simulink model "PV_WIND_BESS_ISLAND_R1"  (R2023b)
settings: Solver=ode14x  StartTime=0.0  StopTime=3.2  FixedStep=25e-6  MaxStep=1e-5  RelTol=1e-3
InitFcn:
  | setup_v2_paths;init_grid_supported_integration;run(which('init_bess_vsm_r10.m'));
undefined symbols (not defined in the file): Base, Control, Converter, DiscIntNeverNeededParam, Drive, Filter, G, PMSG, V2, Wind
libraries: nesl_utility x51, ee_lib x44, fl_lib x25, simulink x6
(part 4 of 4)

== system PV_WIND_BESS_ISLAND_R1/PV Resource/04 Local GFL Control/03 Vdc and Q to current reference/DC Voltage PI ==
  error : Inport
  Integral Derivative : Sum
  Integrator : DiscreteIntegrator  SampleTime=100e-6  ICPrevOutput=DiscIntNeverNeededParam  ICPrevScaledInput=DiscIntNeverNeededParam
  Kaw : Gain  Gain=V2.PV.dynamic.dc_Kaw
  Ki : Gain  Gain=V2.PV.dynamic.dc_Ki_ApVs
  Kp : Gain  Gain=V2.PV.dynamic.dc_Kp_ApV
  Limit : Saturate  UpperLimit=V2.PV.control.Ilimit_peak_A  LowerLimit=-V2.PV.control.Ilimit_peak_A
  Tracking Error : Sum  Inputs=+-
  Unsaturated : Sum
  output : Outport
  wires:
  Tracking Error/1 -> Kaw/1
  Limit/1 -> Tracking Error/1, output/1
  Unsaturated/1 -> Tracking Error/2, Limit/1
  Kp/1 -> Unsaturated/1
  Integrator/1 -> Unsaturated/2
  Integral Derivative/1 -> Integrator/1
  Kaw/1 -> Integral Derivative/2
  Ki/1 -> Integral Derivative/1
  error/1 -> Ki/1, Kp/1

== system PV_WIND_BESS_ISLAND_R1/Wind Resource/02 PMSG dq Machine and Average MSC/01 Torque and Current References/Dispatch Torque Limit ==
  In1 : Inport
  In2 : Inport  Port=2
  Dispatch Inputs : Mux
  Dispatch Torque Cap : Fcn  Expr=0.5*(u(1)+u(2)/u(3)-abs(u(1)-u(2)/u(3)))*u(4)
  Speed Floor : Saturate  UpperLimit=inf  LowerLimit=PMSG.speed_floor_rad_s
  Out1 : Outport
  wires:
  Speed Floor/1 -> Dispatch Inputs/3
  In2/1 -> Dispatch Inputs/1
  Dispatch Inputs/1 -> Dispatch Torque Cap/1
  [WIND_R4__DISPATCH_W] -> Dispatch Inputs/2
  Dispatch Torque Cap/1 -> Out1/1
  In1/1 -> Speed Floor/1
  [WIND_R4__ENABLE] -> Dispatch Inputs/4

== system PV_WIND_BESS_ISLAND_R1/Wind Resource/03 DC Link and Two-Level GSC/Converter AC Measurement/Line Voltage Calculation ==
  Vabc : Inport
  Separate abc : Demux  Outputs=3
  Vab = Va - Vb : Sum  Inputs=+-
  Vab Vbc Vca : Mux  Inputs=3
  Vbc = Vb - Vc : Sum  Inputs=+-
  Vca = Vc - Va : Sum  Inputs=+-
  Vll : Outport
  wires:
  Vabc/1 -> Separate abc/1
  Separate abc/1 -> Vab = Va - Vb/1, Vca = Vc - Va/2
  Separate abc/2 -> Vab = Va - Vb/2, Vbc = Vb - Vc/1
  Separate abc/3 -> Vbc = Vb - Vc/2, Vca = Vc - Va/1
  Vab = Va - Vb/1 -> Vab Vbc Vca/1
  Vbc = Vb - Vc/1 -> Vab Vbc Vca/2
  Vca = Vc - Va/1 -> Vab Vbc Vca/3
  Vab Vbc Vca/1 -> Vll/1  "Vll_inv"

== system PV_WIND_BESS_ISLAND_R1/Wind Resource/04 GFL Control and SPWM/01 Measurements and dq/Current alpha beta to dq ==
  alpha beta : Inport
  theta : Inport  Port=2
  Separate alpha beta : Demux  Outputs=2
  alpha cos : Product
  alpha sin : Product
  beta cos : Product
  beta sin : Product
  cos theta : Trigonometry  Operator=cos
  d = alpha cos + beta sin : Sum
  dq vector : Mux  Inputs=2
  q = -alpha sin + beta cos : Sum  Inputs=-+
  sin theta : Trigonometry
  dq : Outport
  wires:
  alpha beta/1 -> Separate alpha beta/1
  theta/1 -> cos theta/1, sin theta/1
  Separate alpha beta/1 -> alpha cos/1, alpha sin/1
  cos theta/1 -> alpha cos/2, beta cos/2
  Separate alpha beta/2 -> beta sin/1, beta cos/1
  sin theta/1 -> beta sin/2, alpha sin/2
  alpha cos/1 -> d = alpha cos + beta sin/1
  beta sin/1 -> d = alpha cos + beta sin/2
  alpha sin/1 -> q = -alpha sin + beta cos/1
  beta cos/1 -> q = -alpha sin + beta cos/2
  d = alpha cos + beta sin/1 -> dq vector/1
  q = -alpha sin + beta cos/1 -> dq vector/2
  dq vector/1 -> dq/1

== system PV_WIND_BESS_ISLAND_R1/Wind Resource/04 GFL Control and SPWM/01 Measurements and dq/Voltage alpha beta to dq ==
  alpha beta : Inport
  theta : Inport  Port=2
  Separate alpha beta : Demux  Outputs=2
  alpha cos : Product
  alpha sin : Product
  beta cos : Product
  beta sin : Product
  cos theta : Trigonometry  Operator=cos
  d = alpha cos + beta sin : Sum
  dq vector : Mux  Inputs=2
  q = -alpha sin + beta cos : Sum  Inputs=-+
  sin theta : Trigonometry
  dq : Outport
  wires:
  alpha beta/1 -> Separate alpha beta/1
  theta/1 -> cos theta/1, sin theta/1
  Separate alpha beta/1 -> alpha cos/1, alpha sin/1
  cos theta/1 -> alpha cos/2, beta cos/2
  Separate alpha beta/2 -> beta sin/1, beta cos/1
  sin theta/1 -> beta sin/2, alpha sin/2
  alpha cos/1 -> d = alpha cos + beta sin/1
  beta sin/1 -> d = alpha cos + beta sin/2
  alpha sin/1 -> q = -alpha sin + beta cos/1
  beta cos/1 -> q = -alpha sin + beta cos/2
  d = alpha cos + beta sin/1 -> dq vector/1
  q = -alpha sin + beta cos/1 -> dq vector/2
  dq vector/1 -> dq/1

== system PV_WIND_BESS_ISLAND_R1/Wind Resource/04 GFL Control and SPWM/02 Synchronization SRF-PLL/PCC Voltage Prefilter ==
  abc raw : Inport
  Filtered abc : Mux  Inputs=3
  Phase A LPF : TransferFcn  Numerator=[2*pi*Control.PLL.VoltagePrefilterHz]  Denominator=[1 2*pi*Control.PLL.VoltagePrefilterHz]
  Phase B LPF : TransferFcn  Numerator=[2*pi*Control.PLL.VoltagePrefilterHz]  Denominator=[1 2*pi*Control.PLL.VoltagePrefilterHz]
  Phase C LPF : TransferFcn  Numerator=[2*pi*Control.PLL.VoltagePrefilterHz]  Denominator=[1 2*pi*Control.PLL.VoltagePrefilterHz]
  Separate abc : Demux  Outputs=3
  abc filtered : Outport
  wires:
  Separate abc/1 -> Phase A LPF/1
  Phase A LPF/1 -> Filtered abc/1
  Separate abc/2 -> Phase B LPF/1
  Phase B LPF/1 -> Filtered abc/2
  Separate abc/3 -> Phase C LPF/1
  Phase C LPF/1 -> Filtered abc/3
  abc raw/1 -> Separate abc/1
  Filtered abc/1 -> abc filtered/1

== system PV_WIND_BESS_ISLAND_R1/Wind Resource/04 GFL Control and SPWM/02 Synchronization SRF-PLL/Park Voltage ==
  alpha beta : Inport
  theta : Inport  Port=2
  Separate alpha beta : Demux  Outputs=2
  alpha cos : Product
  alpha sin : Product
  beta cos : Product
  beta sin : Product
  cos theta : Trigonometry  Operator=cos
  d = alpha cos + beta sin : Sum
  dq vector : Mux  Inputs=2
  q = -alpha sin + beta cos : Sum  Inputs=-+
  sin theta : Trigonometry
  dq : Outport
  wires:
  alpha beta/1 -> Separate alpha beta/1
  theta/1 -> cos theta/1, sin theta/1
  Separate alpha beta/1 -> alpha cos/1, alpha sin/1
  cos theta/1 -> alpha cos/2, beta cos/2
  Separate alpha beta/2 -> beta sin/1, beta cos/1
  sin theta/1 -> beta sin/2, alpha sin/2
  alpha cos/1 -> d = alpha cos + beta sin/1
  beta sin/1 -> d = alpha cos + beta sin/2
  alpha sin/1 -> q = -alpha sin + beta cos/1
  beta cos/1 -> q = -alpha sin + beta cos/2
  d = alpha cos + beta sin/1 -> dq vector/1
  q = -alpha sin + beta cos/1 -> dq vector/2
  dq vector/1 -> dq/1

== system PV_WIND_BESS_ISLAND_R1/Wind Resource/04 GFL Control and SPWM/03 DC Voltage and Current Reference/Park Voltage ==
  alpha beta : Inport
  theta : Inport  Port=2
  Separate alpha beta : Demux  Outputs=2
  alpha cos : Product
  alpha sin : Product
  beta cos : Product
  beta sin : Product
  cos theta : Trigonometry  Operator=cos
  d : Sum
  dq vector : Mux  Inputs=2
  q : Sum  Inputs=-+
  sin theta : Trigonometry
  dq : Outport
  wires:
  alpha beta/1 -> Separate alpha beta/1
  theta/1 -> cos theta/1, sin theta/1
  Separate alpha beta/1 -> alpha cos/1, alpha sin/1
  cos theta/1 -> alpha cos/2, beta cos/2
  Separate alpha beta/2 -> beta sin/1, beta cos/1
  sin theta/1 -> beta sin/2, alpha sin/2
  alpha cos/1 -> d/1
  beta sin/1 -> d/2
  alpha sin/1 -> q/1
  beta cos/1 -> q/2
  d/1 -> dq vector/1
  q/1 -> dq vector/2
  dq vector/1 -> dq/1

== system PV_WIND_BESS_ISLAND_R1/Wind Resource/04 GFL Control and SPWM/05 dq Current Controller/Inverse Park and Clarke ==
  dq : Inport
  theta : Inport  Port=2
  Inverse Clarke : Gain  Gain=sqrt(2/3)*[1 -0.5 -0.5;0 sqrt(3)/2 -sqrt(3)/2]  Multiplication=Matrix(u*K)
  Separate dq : Demux  Outputs=2
  alpha : Sum  Inputs=+-
  alpha beta : Mux  Inputs=2
  beta : Sum
  cos theta : Trigonometry  Operator=cos
  d cos : Product
  d sin : Product
  q cos : Product
  q sin : Product
  sin theta : Trigonometry
  abc : Outport
  wires:
  dq/1 -> Separate dq/1
  theta/1 -> cos theta/1, sin theta/1
  Separate dq/1 -> d cos/1, d sin/1
  cos theta/1 -> d cos/2, q cos/2
  Separate dq/2 -> q sin/1, q cos/1
  sin theta/1 -> q sin/2, d sin/2
  d cos/1 -> alpha/1
  q sin/1 -> alpha/2
  d sin/1 -> beta/1
  q cos/1 -> beta/2
  alpha/1 -> alpha beta/1
  beta/1 -> alpha beta/2
  alpha beta/1 -> Inverse Clarke/1
  Inverse Clarke/1 -> abc/1

== system PV_WIND_BESS_ISLAND_R1/Wind Resource/04 GFL Control and SPWM/05 dq Current Controller/Park Current ==
  alpha beta : Inport
  theta : Inport  Port=2
  Separate alpha beta : Demux  Outputs=2
  alpha cos : Product
  alpha sin : Product
  beta cos : Product
  beta sin : Product
  cos theta : Trigonometry  Operator=cos
  d : Sum
  dq vector : Mux  Inputs=2
  q : Sum  Inputs=-+
  sin theta : Trigonometry
  dq : Outport
  wires:
  alpha beta/1 -> Separate alpha beta/1
  theta/1 -> cos theta/1, sin theta/1
  Separate alpha beta/1 -> alpha cos/1, alpha sin/1
  cos theta/1 -> alpha cos/2, beta cos/2
  Separate alpha beta/2 -> beta sin/1, beta cos/1
  sin theta/1 -> beta sin/2, alpha sin/2
  alpha cos/1 -> d/1
  beta sin/1 -> d/2
  alpha sin/1 -> q/1
  beta cos/1 -> q/2
  d/1 -> dq vector/1
  q/1 -> dq vector/2
  dq vector/1 -> dq/1

== system PV_WIND_BESS_ISLAND_R1/Wind Resource/04 GFL Control and SPWM/05 dq Current Controller/Park Voltage ==
  alpha beta : Inport
  theta : Inport  Port=2
  Separate alpha beta : Demux  Outputs=2
  alpha cos : Product
  alpha sin : Product
  beta cos : Product
  beta sin : Product
  cos theta : Trigonometry  Operator=cos
  d : Sum
  dq vector : Mux  Inputs=2
  q : Sum  Inputs=-+
  sin theta : Trigonometry
  dq : Outport
  wires:
  alpha beta/1 -> Separate alpha beta/1
  theta/1 -> cos theta/1, sin theta/1
  Separate alpha beta/1 -> alpha cos/1, alpha sin/1
  cos theta/1 -> alpha cos/2, beta cos/2
  Separate alpha beta/2 -> beta sin/1, beta cos/1
  sin theta/1 -> beta sin/2, alpha sin/2
  alpha cos/1 -> d/1
  beta sin/1 -> d/2
  alpha sin/1 -> q/1
  beta cos/1 -> q/2
  d/1 -> dq vector/1
  q/1 -> dq vector/2
  dq vector/1 -> dq/1

== system PV_WIND_BESS_ISLAND_R1/PV Resource/02 MPPT Boost and DC Link/MPPT and Curtailment/02 Dispatch curtailment/Curtailment PI ==
  error : Inport
  Integral Derivative : Sum
  Integrator : DiscreteIntegrator  InitialCondition=min(180,V2.PV.dynamic.Vpv_max_V-V2.PV.dynamic.Vmp_initial_V)  SampleTime=100e-6  ICPrevOutput=DiscIntNeverNeededParam  ICPrevScaledInput=DiscIntNeverNeededParam
  Kaw : Gain  Gain=30
  Ki : Gain  Gain=V2.PV.dynamic.curtail_Ki_VpWs
  Kp : Gain  Gain=V2.PV.dynamic.curtail_Kp_VpW
  Limit : Saturate  UpperLimit=400  LowerLimit=0
  Tracking Error : Sum  Inputs=+-
  Unsaturated : Sum
  output : Outport
  wires:
  Tracking Error/1 -> Kaw/1
  Limit/1 -> Tracking Error/1, output/1
  Unsaturated/1 -> Tracking Error/2, Limit/1
  Kp/1 -> Unsaturated/1
  Integrator/1 -> Unsaturated/2
  Integral Derivative/1 -> Integrator/1
  Kaw/1 -> Integral Derivative/2
  Ki/1 -> Integral Derivative/1
  error/1 -> Ki/1, Kp/1

== system PV_WIND_BESS_ISLAND_R1/PV Resource/02 MPPT Boost and DC Link/MPPT and Curtailment/04 Boost duty regulator/Boost Voltage PI ==
  error : Inport
  Integral Derivative : Sum
  Integrator : DiscreteIntegrator  InitialCondition=0.4  SampleTime=100e-6  ICPrevOutput=DiscIntNeverNeededParam  ICPrevScaledInput=DiscIntNeverNeededParam
  Kaw : Gain  Gain=V2.PV.dynamic.boost_Kaw
  Ki : Gain  Gain=V2.PV.dynamic.boost_Ki
  Kp : Gain  Gain=V2.PV.dynamic.boost_Kp
  Limit : Saturate  UpperLimit=V2.PV.dynamic.duty_max  LowerLimit=V2.PV.dynamic.duty_min
  Tracking Error : Sum  Inputs=+-
  Unsaturated : Sum
  output : Outport
  wires:
  Tracking Error/1 -> Kaw/1
  Limit/1 -> Tracking Error/1, output/1
  Unsaturated/1 -> Tracking Error/2, Limit/1
  Kp/1 -> Unsaturated/1
  Integrator/1 -> Unsaturated/2
  Integral Derivative/1 -> Integrator/1
  Kaw/1 -> Integral Derivative/2
  Ki/1 -> Integral Derivative/1
  error/1 -> Ki/1, Kp/1

== matlab function PV_WIND_BESS_ISLAND_R1/BESS Synchronism and Dispatch/Synchrocheck and latch ==
  data: u input; y output; z input; z1 output
function [y,z1]=bw_sync_kernel(u,z)
% 1 ms commissioning supervisor. No grid angle is exported to the VSM.
% vectors: BESS phase-ground, grid phase-ground, external P/Q, time,
% permit, actual Q. Voltage trim is in LV line-line RMS volts.
u=reshape(u,11,1);z=reshape(z,9,1);T=.001;
v=u(1:3);g=u(4:6);tm=u(9);
a=(2*v(1)-v(2)-v(3))/3;b=(v(2)-v(3))/sqrt(3);
c=(2*g(1)-g(2)-g(3))/3;d=(g(2)-g(3))/sqrt(3);
vb=hypot(a,b)*sqrt(1.5)/1e4;vg=hypot(c,d)*sqrt(1.5)/1e4;
th=atan2(b,a);tg=atan2(d,c);err=atan2(sin(tg-th),cos(tg-th));
fb=z(3)+.12*(atan2(sin(th-z(1)),cos(th-z(1)))/(2*pi*T)-z(3));
fg=z(4)+.12*(atan2(sin(tg-z(2)),cos(tg-z(2)))/(2*pi*T)-z(4));
ok=tm>.15 && vb>.9 && vb<1.1 && vg>.9 && vg<1.1 && ...
    fb>48 && fb<52 && fg>48 && fg<52 && abs(fb-fg)<.06 && ...
    abs(vb-vg)<.015 && abs(err)<2*pi/180;
dwell=0;if ok && u(10)>.5,dwell=z(5)+T;end
closed=z(6)>.5 || dwell>=.05;
trim=z(7);pref=z(8);qref=z(9);syncW=0;
if ~closed
 if tm>.12 && vb>.5
  syncW=max(-4e6,min(4e6,5e6*100/50*1.2*err)); % swing torque, not phase overwrite
  trim=trim+T*900*(vg-vb);
 end
else
 pref=pref+max(-8e6*T,min(8e6*T,u(7)-pref));
 qref=qref+max(-3e6*T,min(3e6*T,u(8)-qref));
 trim=trim+T*8e-5*(qref-u(11));
end
% LV voltage-drop compensation: (R*P+X*Q)/Vll, plus the local Q droop.
% 0.20 pu R and 0.23 pu net X on 690 V / 6.25 MVA commissioning base.
ff=(.20*pref+.23*qref)*690/6.25e6+.05*690/5e6*qref;
trim=max(-65-ff,min(65-ff,trim));z1=[th;tg;fb;fg;dwell;double(closed);trim;pref;qref];
y=[1-double(closed);pref+syncW;trim+ff;vb;vg;err*180/pi;fb;fg;dwell;double(ok);pref];
end

== matlab function PV_WIND_BESS_ISLAND_R1/02 GFM PCS and Step-up/04 PCS Filter and Transformer/Measured voltage and current loops/Cascaded dq regulation ==
  data: u input; m output; z input; k input; znew output; diag output
function [m,znew,diag]=bess_r9_ac_kernel(u,z,k)
%#codegen
% Input vectors are instantaneous phase quantities, not RMS or PCC P/Q.
% Voltage measured at the LCL shunt node; current measured before L1.
u=reshape(u,13,1);z=reshape(z,4,1);ref=u(1:3); vc=u(4:6); i1=u(7:9); i2=u(10:12); vdc=max(u(13),100);
T=k(1); L=k(2); R=k(3); C=k(4); wi=k(5); wv=k(6); imax=k(7); mm=k(8);
w=k(9); amp=max(sqrt(2/3*(ref.'*ref)),1e-8);
sn=ref/amp; cs=[sn(3)-sn(2);sn(1)-sn(3);sn(2)-sn(1)]/sqrt(3);
F=(2/3)*[sn.';cs.']; invF=[sn cs]; J=[0 -1;1 0];
v=F*vc; i=F*i1; ig=F*i2; vr=[min(amp,mm)*vdc/2;0];
if numel(k)>9,vr=vr*k(10);end % R10 AC build-up; oscillator coordinates stay valid.
% Optional grid-parallel adapter. A positive-real vector output impedance
% opposes circulating current in both axes; standalone R9/R10 omit it.
if numel(k)>11,vr=vr-k(12)*ig-k(13)*J*ig;end
ev=vr-v; kv=1.414*C*wv; ki=C*wv^2;
ir0=ig+w*C*J*v+kv*ev+z(1:2);
fi=min(1,imax/max(norm(ir0),1e-9)); ir=fi*ir0;
% GFM feedforward must establish voltage even with a discharged filter.
% Capacitor-current feedback adds active damping to the LCL mode.
ei=ir-i; raw=vr+R*i+w*L*J*i+L*wi*ei+z(3:4)-0.3*L*wi*(i-ig-w*C*J*v);
requested=raw;
if numel(k)>9
 % Predominantly use measured capacitor voltage as current-loop feedforward.
 % A small command feedforward remains for excitation of the initially dead bus.
 raw=raw+.85*(v-vr);requested=raw;
 % Project a short-horizon L1 current prediction into a guarded circle.
 % Inverse inductor equation maps the feasible current back to bridge volts.
 holdV=v+R*i+w*L*J*i;horizon=3*T;
 predicted=i+horizon/L*(raw-holdV);
 factor=min(1,k(11)*imax/max(norm(predicted),1e-9));
 raw=holdV+(L/horizon)*(factor*predicted-i);
end
fv=min(1,mm*vdc/(2*max(norm(raw),1e-9))); applied=fv*raw;
znew=z+T*[ki*ev+wv*(ir-ir0);R*wi*ei+wi*(applied-requested)];
m=2/vdc*invF*applied;
diag=[norm(ir0);norm(ir);norm(i);fi;fv;norm(v);norm(vr)];
end
